simulink model "untitled_restored_from_autosave"  (R2026a)
settings: Solver=FixedStepAuto  FixedStep=.001
libraries: cstblocks_lti x2
settings Model: Creator=ms110  LastModifiedBy=ms110

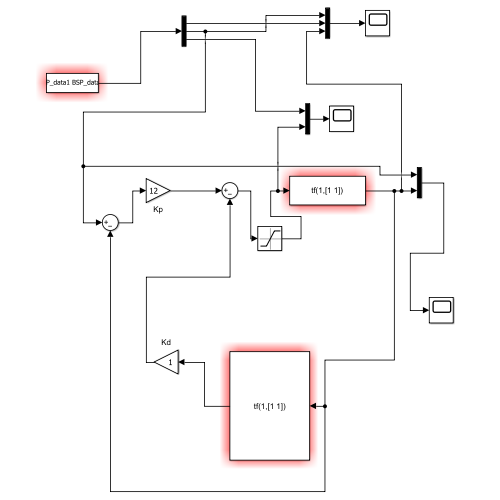
[thumbnail: Simulink's stored preview of the top-level diagram]
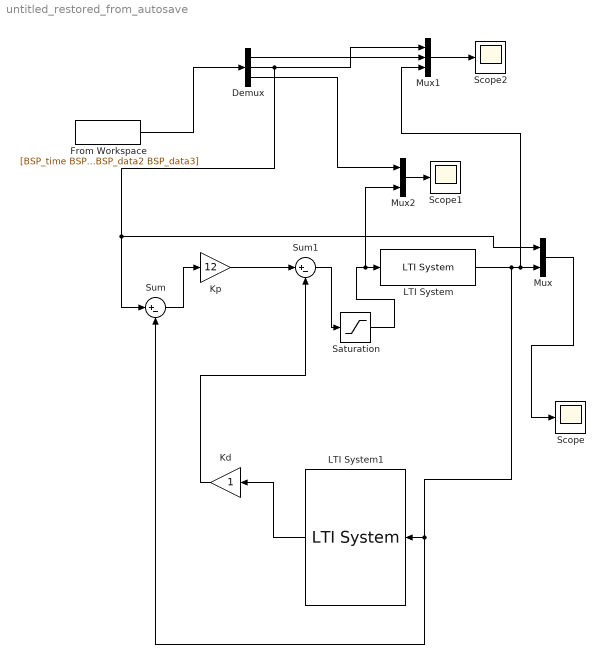
== system untitled_restored_from_autosave ==
  Demux : Demux  Outputs=3
  From Workspace : FromWorkspace  VariableName=[BSP_time BSP_data1 BSP_data2 BSP_data3]
  Kd : Gain
  Kp : Gain  Gain=12
  LTI System : cstblocks_lti/LTI System  sys=pos_func_d  IC=[]  PadeOrder=0
      settings: LibrarySourceBlock=cstblocks/LTI System
  LTI System1 : cstblocks_lti/LTI System  sys=tust_prox  IC=[]  PadeOrder=0
      settings: LibrarySourceBlock=cstblocks/LTI System
  Mux : Mux  Inputs=2
  Mux1 : Mux  Inputs=3
  Mux2 : Mux  Inputs=2
  Saturation : Saturate  UpperLimit=10  LowerLimit=-10
  Scope : Scope
      settings: ActiveDisplayYMinimum=0.71865715444513423  ActiveDisplayYMaximum=1.1503006909988887
  Scope1 : Scope
      settings: ActiveDisplayYMinimum=-1  ActiveDisplayYMaximum=1
  Scope2 : Scope
      settings: ActiveDisplayYMinimum=-1  ActiveDisplayYMaximum=1  DataLoggingVariableName=ScopeData2
  Sum : Sum  Inputs=|+-
  Sum1 : Sum  Inputs=|+-
  wires:
  Kp/1 -> Sum1/1
  LTI System/1 -> Mux1/3, Mux/2, Sum/2, LTI System1/1
  LTI System1/1 -> Kd/1
  Kd/1 -> Sum1/2
  Sum/1 -> Kp/1
  Mux/1 -> Scope/1
  Sum1/1 -> Saturation/1
  Saturation/1 -> Mux2/2, LTI System/1
  From Workspace/1 -> Demux/1
  Demux/2 -> Mux1/1, Mux/1, Sum/1
  Demux/1 -> Mux1/2
  Mux1/1 -> Scope2/1
  Mux2/1 -> Scope1/1
  Demux/3 -> Mux2/1
